simulink model "Simulink_2_Motor_Con_Control"  (R2023a)
settings: Solver=ode45  StartTime=0.0  StopTime=1.5  MaxStep=0.002  RelTol=1e-3
settings Model: Creator=juanj  LastModifiedBy=juanj
settings RTWCC: GPUComputeCapability=5.0
settings ConfigComp: CovBoundaryAbsTol=1.0e-5

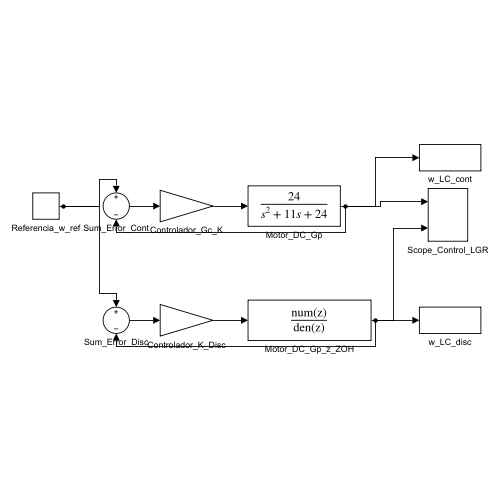
[thumbnail: Simulink's stored preview of the top-level diagram]
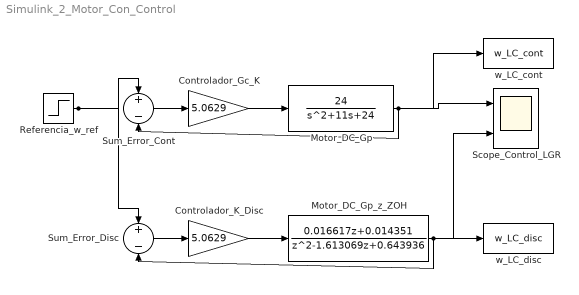
== system Simulink_2_Motor_Con_Control ==
  Controlador_Gc_K : Gain  Gain=5.0629
  Controlador_K_Disc : Gain  Gain=5.0629  SampleTime=0.04
  Motor_DC_Gp : TransferFcn  Numerator=[24]  Denominator=[1 11 24]
  Motor_DC_Gp_z_ZOH : DiscreteTransferFcn  Numerator=[0.016617 0.014351]  Denominator=[1 -1.613069 0.643936]  SampleTime=0.04
  Referencia_w_ref : Step  Time=0  SampleTime=0
  Scope_Control_LGR : Scope  NumInputPorts=2
  Sum_Error_Cont : Sum  Inputs=+-
  Sum_Error_Disc : Sum  Inputs=+-
  w_LC_cont : ToWorkspace  VariableName=w_LC_cont  SaveFormat=Timeseries  SampleTime=-1
  w_LC_disc : ToWorkspace  VariableName=w_LC_disc  SaveFormat=Timeseries  SampleTime=-1
  wires:
  Referencia_w_ref/1 -> Sum_Error_Cont/1, Sum_Error_Disc/1
  Sum_Error_Cont/1 -> Controlador_Gc_K/1
  Controlador_Gc_K/1 -> Motor_DC_Gp/1
  Motor_DC_Gp/1 -> Scope_Control_LGR/1, w_LC_cont/1, Sum_Error_Cont/2
  Sum_Error_Disc/1 -> Controlador_K_Disc/1
  Controlador_K_Disc/1 -> Motor_DC_Gp_z_ZOH/1
  Motor_DC_Gp_z_ZOH/1 -> Scope_Control_LGR/2, w_LC_disc/1, Sum_Error_Disc/2
